simulink model "topology"  (R2024b)
settings: Solver=FixedStepDiscrete  StartTime=0.0  StopTime=0.2  FixedStep=1e-6  MaxStep=1e-6  RelTol=1e-6
libraries: spsMosfetLib x16, spsSeriesRLCBranchLib x16, spsIdealSwitchLib x10, simulink x7, spsVoltageMeasurementLib x6, spsCurrentMeasurementLib x5, spsDCVoltageSourceLib x4, spsACVoltageSourceLib x1, sps_lib x1
settings Model: DataDictionary=CHB_Data.sldd  Creator=licuiting  LastModifiedBy=licuiting
settings SolverCC: InitialStep=1e-6
settings ModelReferenceCC: ModelReferenceNumInstancesAllowed=Single

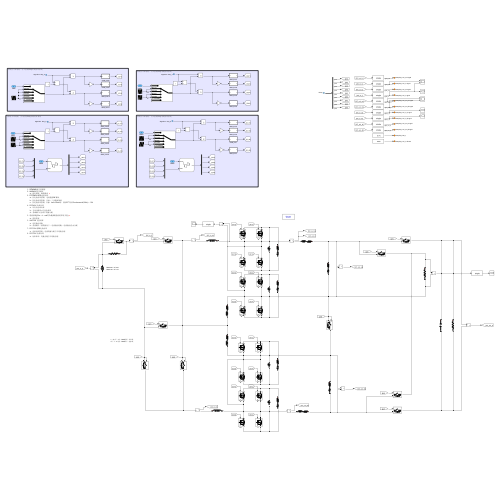
[thumbnail: Simulink's stored preview of the top-level diagram]
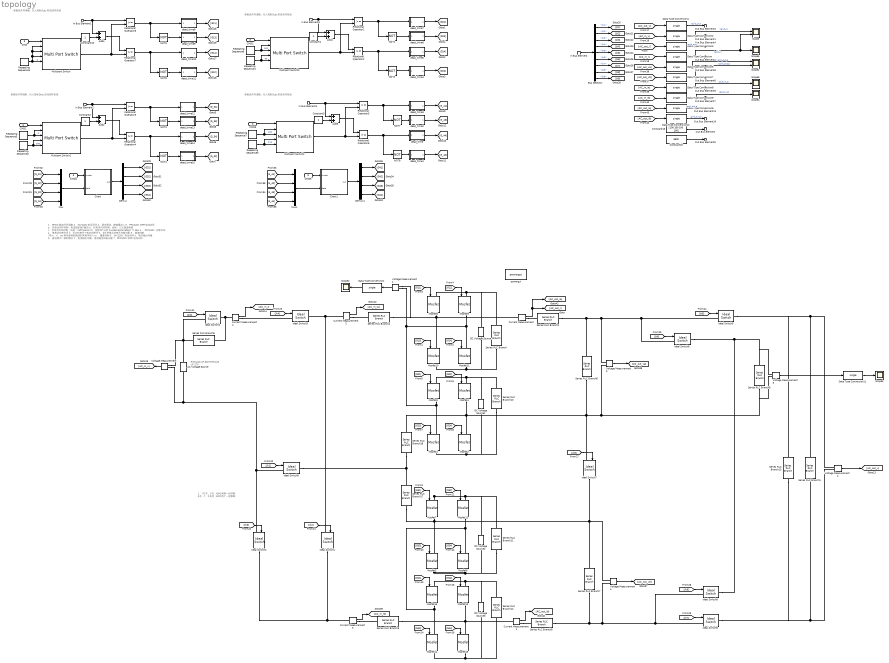
== system topology ==
  note: RMS:240   UF:340
      | RMS:120   UF:170
  note: 1、SPWM载波开环调制
      | 2、INV240V电压闭环
      | a、逐步限流、峰值限流 x
      | 3、PFC240V QPR电流内环
      | a、仅电流内环控制：电流超前90°解决
      | b、仅电流内环控制：目标：三次谐波削弱
      | c、仅电流内环控制：目标：Iref=15cos时，实际FFT分析 Fundamental(50Hz) = 15A
      | 4、PFC240V 功率外环
      | a、单有功功率外环
      | b、无功功率环+有功功率环
      | d、各H桥单元功率不均衡分配
      | 5、谐波抑制 (带rc、rl、rcd等负载抑制谐波的常用手段) x
      | a、 重复控制
      | 6、INV120V 电压闭环
      | a、电压输出均衡
      | b、直流源不一致的情况下，电流输出均衡，电流输出自由分配
      | 7、PFC120V QPR电流内环
      | a、电流内环控制，电流均衡分配与不均衡分配
      | 8、PFC120V 功率外环
      | a、功率外环，均衡分配与不均衡分配
  note: 1、2打开，3关，BMS两两一组并联
      | 3开，1、2关闭，BMS四个一起串联
  note: 单极性开环调制，引入控制Duty形成闭环系统
  note: 单极性开环调制，引入控制Duty形成闭环系统
  note: 单极性开环调制，引入控制Duty形成闭环系统
  note: 单极性开环调制，引入控制Duty形成闭环系统
  In Bus Element : Inport  PortName=Relay
  In Bus Element1 : Inport  Port=2  PortName=Algorithm  Element=duty_a
  In Bus Element3 : Inport  Port=2  PortName=Algorithm  Element=duty_a
  In Bus Element2 : Inport  Port=2  PortName=Algorithm  Element=duty_b
  In Bus Element4 : Inport  Port=2  PortName=Algorithm  Element=duty_b
  CMD : Inport  Port=3  OutDataTypeStr=Enum: CHB_MODE
  AC Voltage Source : spsACVoltageSourceLib/AC Voltage Source  Amplitude=170  Phase=0  Frequency=50  SampleTime=0  Measurements=None  BusType=swing  Pref=10e3  Qref=0  Qmin=-inf  Qmax=+inf
  Add{1..4} (4 alike) : Sum
  Bus Selector : BusSelector  OutputSignals=jk1,jk2,jk3,jk4,jk5,jk6,jk7,jk8,jk9
  CMD{1..5} (5 alike) : InportShadow  Port=3  OutDataTypeStr=Enum: CHB_MODE
  Chart : Stateflow chart  TreatAsAtomicUnit=on
  Chart1 : Stateflow chart  TreatAsAtomicUnit=on
  Constant{1..3,10} (4 alike) : Constant
  Constant16 : Constant  Value=[100 100 100 100]  OutDataTypeStr=single
  Constant20 : Constant  Value=3600  OutDataTypeStr=single
  Current Measurement{,1..4} (5 alike) : spsCurrentMeasurementLib/Current Measurement  PhasorSimulation=off  OutputType=Complex  PSBequivalent=0
  DC Voltage Source{,1..3} (4 alike) : spsDCVoltageSourceLib/DC Voltage Source  Amplitude=100  Measurements=None
  Data Type Conversion{,1..11} (12 alike) : DataTypeConversion  OutDataTypeStr=single  SaturateOnIntegerOverflow=off  RndMeth=Floor
  Demux : Demux
  Demux1 : Demux
  Ideal Switch{0..9} (10 alike) : spsIdealSwitchLib/Ideal Switch  Ron=0.001  Lon=0  IC=0  Rs=1e5  Cs=inf  Measurements=off
  Mosfet{1..16} (16 alike) : spsMosfetLib/Mosfet  Ron=0.01  Lon=0  Rd=0.01  Vfd=0  IC=0  Rs=1e5  Cs=inf  Measurements=on
  Multiport Switch{,1..3} (4 alike) : MultiPortSwitch  DataPortOrder=Specify indices  Inputs=4  DataPortIndices={CHB_MODE.INV120,CHB_MODE.PFC120,CHB_MODE.INV240,CHB_MODE.PFC240,CHB_MODE.STANDBY}  OutDataTypeStr=single  SaturateOnIntegerOverflow=off  InputSameDT=off
  Mux : Mux
  Mux1 : Mux
  NOT{1..8} (8 alike) : Logic  Operator=NOT  IconShape=distinctive  AllPortsSameDT=off  OutDataTypeStr=boolean
  Relational Operator{1..8} (8 alike) : RelationalOperator  OutDataTypeStr=boolean  RndMeth=Simplest  InputSameDT=off
  Repeating Sequence1 : simulink/Sources/Repeating Sequence  rep_seq_t=[0 2.5e-5 7.5e-5 1e-4]  rep_seq_y=[0.5 1 0 0.5]
  Repeating Sequence2 : simulink/Sources/Repeating Sequence  rep_seq_t=[0 5e-5 1e-4]  rep_seq_y=[0 1 0]
  Repeating Sequence3 : simulink/Sources/Repeating Sequence  rep_seq_t=[0 2.5e-5 7.5e-5 1e-4]  rep_seq_y=[0.5 0 1 0.5]
  Repeating Sequence4 : simulink/Sources/Repeating Sequence  rep_seq_t=[0 5e-5 1e-4]  rep_seq_y=[1 0 1]
  Repeating Sequence5 : simulink/Sources/Repeating Sequence  rep_seq_t=[0 5e-5 1e-4]  rep_seq_y=[1 0 1]
  Repeating Sequence6 : simulink/Sources/Repeating Sequence  rep_seq_t=[0 5e-5 1e-4]  rep_seq_y=[0 1 0]
  Repeating Sequence7 : simulink/Sources/Repeating Sequence  rep_seq_t=[0 5e-5 1e-4]  rep_seq_y=[0 1 0]
  Scope : Scope  NumInputPorts=2
  Scope1 : Scope  NumInputPorts=2
  Scope{2..6} (5 alike) : Scope
  Series RLC Branch{,10..12} (4 alike) : spsSeriesRLCBranchLib/Series RLC Branch  LConnTagsString=__new0  RConnTagsString=__new0  BranchType=RC  Resistance=0.5  Inductance=1e-3  SetiL0=off  InitialCurrent=0  Capacitance=4.7e-6  Setx0=off  InitialVoltage=0  Measurements=None
  Series RLC Branch1 : spsSeriesRLCBranchLib/Series RLC Branch  LConnTagsString=__new0  RConnTagsString=__new0  BranchType=R  Resistance=100  Inductance=1e-3  SetiL0=off  InitialCurrent=0  Capacitance=1e-6  Setx0=off  InitialVoltage=0  Measurements=None
  Series RLC Branch13 : spsSeriesRLCBranchLib/Series RLC Branch  LConnTagsString=__new0  RConnTagsString=__new0  BranchType=C  Resistance=100  Inductance=1e-3  SetiL0=off  InitialCurrent=0  Capacitance=4.2e-6  Setx0=off  InitialVoltage=0  Measurements=None
  Series RLC Branch{2,9,17..18} (4 alike) : spsSeriesRLCBranchLib/Series RLC Branch  LConnTagsString=__new0  RConnTagsString=__new0  BranchType=RL  Resistance=0.2  Inductance=1e-3  SetiL0=off  InitialCurrent=0  Capacitance=1e-6  Setx0=off  InitialVoltage=0  Measurements=None
  Series RLC Branch3 : spsSeriesRLCBranchLib/Series RLC Branch  LConnTagsString=__new0  RConnTagsString=__new0  BranchType=L  Resistance=0.2  Inductance=1e-3  SetiL0=off  InitialCurrent=0  Capacitance=1e-6  Setx0=off  InitialVoltage=0  Measurements=None
  Series RLC Branch4 : spsSeriesRLCBranchLib/Series RLC Branch  LConnTagsString=__new0  RConnTagsString=__new0  BranchType=L  Resistance=0.2  Inductance=1e-3  SetiL0=off  InitialCurrent=0  Capacitance=1e-6  Setx0=off  InitialVoltage=0  Measurements=None
  Series RLC Branch5 : spsSeriesRLCBranchLib/Series RLC Branch  LConnTagsString=__new0  RConnTagsString=__new0  BranchType=R  Resistance=0.2  Inductance=2e-3  SetiL0=off  InitialCurrent=0  Capacitance=1e-6  Setx0=off  InitialVoltage=0  Measurements=None
  Series RLC Branch6 : spsSeriesRLCBranchLib/Series RLC Branch  LConnTagsString=__new0  RConnTagsString=__new0  BranchType=RC  Resistance=0.2  Inductance=1e-3  SetiL0=off  InitialCurrent=0  Capacitance=4.2e-6  Setx0=off  InitialVoltage=0  Measurements=None
  Series RLC Branch7 : spsSeriesRLCBranchLib/Series RLC Branch  LConnTagsString=__new0  RConnTagsString=__new0  BranchType=RC  Resistance=0.2  Inductance=1e-3  SetiL0=off  InitialCurrent=0  Capacitance=4.2e-6  Setx0=off  InitialVoltage=0  Measurements=None
  Series RLC Branch8 : spsSeriesRLCBranchLib/Series RLC Branch  LConnTagsString=__new0  RConnTagsString=__new0  BranchType=R  Resistance=5  Inductance=1e-3  SetiL0=off  InitialCurrent=0  Capacitance=1e-6  Setx0=off  InitialVoltage=0  Measurements=None
  Voltage Measurement{,1..5} (6 alike) : spsVoltageMeasurementLib/Voltage Measurement  PhasorSimulation=off  OutputType=Complex  PSBequivalent=0
  dead_time : Subsystem  TreatAsAtomicUnit=on
  dead_time1 : Subsystem  TreatAsAtomicUnit=on
  dead_time10 : Subsystem  TreatAsAtomicUnit=on
  dead_time11 : Subsystem  TreatAsAtomicUnit=on
  dead_time12 : Subsystem  TreatAsAtomicUnit=on
  dead_time13 : Subsystem  TreatAsAtomicUnit=on
  dead_time14 : Subsystem  TreatAsAtomicUnit=on
  dead_time15 : Subsystem  TreatAsAtomicUnit=on
  dead_time2 : Subsystem  TreatAsAtomicUnit=on
  dead_time3 : Subsystem  TreatAsAtomicUnit=on
  dead_time4 : Subsystem  TreatAsAtomicUnit=on
  dead_time5 : Subsystem  TreatAsAtomicUnit=on
  dead_time6 : Subsystem  TreatAsAtomicUnit=on
  dead_time7 : Subsystem  TreatAsAtomicUnit=on
  dead_time8 : Subsystem  TreatAsAtomicUnit=on
  dead_time9 : Subsystem  TreatAsAtomicUnit=on
  powergui : sps_lib/powergui  Priority=1  SimulationMode=Discrete  SampleTime=1e-6  frequency=60  Iterations=50  frequencyindice=0  Pbase=100e6  ErrMax=1e-4  UnitsV=kV  UnitsW=MW  buscounter=0  FunctionMessages=off  echomessages=off  EnableUseOfTLC=off  CurrentSourceSwitches=off  DisableSnubberDevices=off  DisableRonSwitches=off  DisableVfSwitches=off  DisplayEquations=off  AutomaticDiscreteSolvers=off  SolverType=Tustin/Backward Euler (TBE)  Interpol=off  ExternalGateDelay=off  methode=off  Ts=100  x0status=blocks  SPID=on  SwTol=0  HookPort=off  NonlinearTolerance=1e-4  nMaxIteration=100  ContinueOnMaxIteration=off  RestoreLinks=warning  ResistiveCurrentMeasurement=off  Frange=[0:2:500]  Ylog=off  Xlog=on  ShowGrid=off  save=off  variable=ZData  structure=0  ZoomFFT=off  StartTime=0.0  cycles=1  DisplayStyle=1  fundamental=60  FreqAxis=off  MaxFrequency=1000  frequencyindicesteady=1  RmsSteady=1  display=off
  Out Bus Element1 : Outport  PortName=Sampling  Element=AC_in.Vgrid
  Out Bus Element2 : Outport  PortName=Sampling  Element=AC_in.Igrid
  Out Bus Element5 : Outport  PortName=Sampling  Element=AC_in.Power
  Out Bus Element3 : Outport  PortName=Sampling  Element=AC_out.Vgrid
  Out Bus Element4 : Outport  PortName=Sampling  Element=AC_out.Igrid
  Out Bus Element8 : Outport  PortName=Sampling  Element=AC_out_A.Vgrid
  Out Bus Element11 : Outport  PortName=Sampling  Element=AC_out_A.Igrid
  Out Bus Element6 : Outport  PortName=Sampling  Element=AC_out_B.Vgrid
  Out Bus Element10 : Outport  PortName=Sampling  Element=AC_out_B.Igrid
  Out Bus Element9 : Outport  PortName=Sampling  Element=AC_in_A.Igrid
  Out Bus Element7 : Outport  PortName=Sampling  Element=AC_in_B.Igrid
  Out Bus Element : Outport  PortName=Sampling  Element=bat_v
  wires:
  Relational Operator6/1 -> dead_time8/1(Input), NOT5/1
  Add4/1 -> Relational Operator7/1
  Constant10/1 -> Add4/2
  Relational Operator2/1 -> dead_time5/1(Input), NOT2/1
  Constant1/1 -> Add1/2
  Add1/1 -> Relational Operator2/1
  Relational Operator1/1 -> dead_time7/1(Input), NOT1/1
  Relational Operator3/1 -> dead_time12/1(Input), NOT3/1
  Add2/1 -> Relational Operator4/1
  Constant2/1 -> Add2/2
  Relational Operator4/1 -> dead_time14/1(Input), NOT4/1
  Relational Operator8/1 -> dead_time/1(Input), NOT8/1
  Constant3/1 -> Add3/2
  Add3/1 -> Relational Operator8/1
  Relational Operator5/1 -> dead_time3/1(Input), NOT7/1
  [G14] -> Mosfet11/1
  [G13] -> Mosfet10/1
  [G11] -> Mosfet8/1
  [G12] -> Mosfet9/1
  [G21] -> Mosfet3/1
  [G22] -> Mosfet4/1
  [G23] -> Mosfet1/1
  [G24] -> Mosfet2/1
  [G31] -> Mosfet7/1
  [G34] -> Mosfet6/1
  [G41] -> Mosfet16/1
  [G44] -> Mosfet15/1
  Relational Operator7/1 -> dead_time10/1(Input), NOT6/1
  [G33] -> Mosfet5/1
  [G32] -> Mosfet12/1
  [G43] -> Mosfet14/1
  [G42] -> Mosfet13/1
  Data Type Conversion1/1 -> Scope2/1
  Voltage Measurement1/1 -> Data Type Conversion1/1
  Voltage Measurement/1 -> [AC_in_v]
  Current Measurement/1 -> [AC_out_i], [AC_out_ia]
  [AC_out_v] -> Data Type Conversion4/1
  [AC_in_i] -> Data Type Conversion/1
  [AC_in_v] -> Data Type Conversion2/1
  [AC_out_i] -> Data Type Conversion3/1
  In Bus Element/1 -> Bus Selector/1
  Bus Selector/1 -> [jk1]  "<jk1>"
  Bus Selector/2 -> [jk2]  "<jk2>"
  Bus Selector/3 -> [jk3]  "<jk3>"
  Bus Selector/4 -> [jk4]  "<jk4>"
  Bus Selector/5 -> [jk5]  "<jk5>"
  Bus Selector/6 -> [jk6]  "<jk6>"
  Bus Selector/7 -> [jk7]  "<jk7>"
  Bus Selector/8 -> [jk8]  "<jk8>"
  Constant16/1 -> Out Bus Element/1
  Data Type Conversion2/1 -> Scope/1, Out Bus Element1/1  "Vgrid_in"
  Data Type Conversion/1 -> Scope/2, Scope5/1, Out Bus Element2/1  "Igrid_in"
  Data Type Conversion4/1 -> Out Bus Element3/1  "Vgrid_out"
  Data Type Conversion3/1 -> Out Bus Element4/1  "Igrid_out"
  Voltage Measurement2/1 -> [AC_out_v]
  [jk4] -> Ideal Switch3/1
  [jk1] -> Ideal Switch0/1
  [jk3] -> Ideal Switch2/1
  [jk2] -> Ideal Switch1/1
  [jk6] -> Ideal Switch6/1
  [jk8] -> Ideal Switch7/1
  [jk5] -> Ideal Switch5/1
  Constant20/1 -> Out Bus Element5/1
  CMD/1 -> Multiport Switch/1
  Multiport Switch3/1 -> Relational Operator1/2, Relational Operator2/2
  Multiport Switch2/1 -> Relational Operator5/2, Relational Operator8/2
  Multiport Switch/1 -> Relational Operator6/2, Relational Operator7/2
  Repeating Sequence2/1 -> Multiport Switch1/4, Multiport Switch1/5  "180"
  Repeating Sequence4/1 -> Multiport Switch/3, Multiport Switch/2, Multiport Switch/4, Multiport Switch/5  "0"
  Repeating Sequence1/1 -> Multiport Switch3/4, Multiport Switch3/5  "90"
  Repeating Sequence3/1 -> Multiport Switch2/4, Multiport Switch2/5  "270"
  CMD1/1 -> Multiport Switch1/1
  CMD3/1 -> Multiport Switch2/1
  CMD2/1 -> Multiport Switch3/1
  Repeating Sequence5/1 -> Multiport Switch1/2, Multiport Switch1/3  "0"
  Repeating Sequence6/1 -> Multiport Switch3/2, Multiport Switch3/3  "180"
  Repeating Sequence7/1 -> Multiport Switch2/3, Multiport Switch2/2  "180"
  [jk7] -> Ideal Switch9/1
  Bus Selector/9 -> [jk9]  "<jk9>"
  [jk9] -> Ideal Switch8/1
  Multiport Switch1/1 -> Relational Operator3/2, Relational Operator4/2
  [G_34] -> Mux/4
  [G_33] -> Mux/3
  [G_32] -> Mux/2
  [G_31] -> Mux/1
  Mux/1 -> Chart/2(data)
  CMD4/1 -> Chart/1(mode)
  Chart/1(out) -> Demux/1
  Demux/1 -> [G31]
  Demux/2 -> [G32]
  Demux/3 -> [G33]
  Demux/4 -> [G34]
  Mux1/1 -> Chart1/2(data)
  [G_41] -> Mux1/1
  [G_42] -> Mux1/2
  [G_43] -> Mux1/3
  [G_44] -> Mux1/4
  CMD5/1 -> Chart1/1(mode)
  Chart1/1(out) -> Demux1/1
  Demux1/1 -> [G41]
  Demux1/2 -> [G42]
  Demux1/3 -> [G43]
  Demux1/4 -> [G44]
  [AC_out_vb] -> Data Type Conversion7/1
  [AC_out_va] -> Data Type Conversion5/1
  Data Type Conversion7/1 -> Scope1/2, Out Bus Element6/1  "vgrid_out_b"
  Data Type Conversion5/1 -> Scope1/1, Out Bus Element8/1  "vgrid_out_a"
  Data Type Conversion9/1 -> Out Bus Element7/1, Scope4/1  "igrid_in_b"
  Data Type Conversion8/1 -> Out Bus Element9/1, Scope6/1  "igrid_in_a"
  In Bus Element1/1 -> Relational Operator6/1, Add4/1
  In Bus Element3/1 -> Add1/1, Relational Operator1/1
  In Bus Element4/1 -> Add3/1, Relational Operator5/1
  In Bus Element2/1 -> Add2/1, Relational Operator3/1
  [AC_in_ia] -> Data Type Conversion8/1
  [AC_in_ib] -> Data Type Conversion9/1
  Current Measurement2/1 -> [AC_in_ia]
  Current Measurement3/1 -> [AC_in_ib]
  Current Measurement4/1 -> [AC_in_i]
  [jk2] -> Ideal Switch4/1
  Data Type Conversion6/1 -> Out Bus Element11/1  "igrid_out_a"
  Data Type Conversion10/1 -> Out Bus Element10/1  "igrid_out_b"
  [AC_out_ia] -> Data Type Conversion6/1
  [AC_out_ib] -> Data Type Conversion10/1
  Current Measurement1/1 -> [AC_out_ib]
  Voltage Measurement3/1 -> [AC_out_va]
  Voltage Measurement4/1 -> [AC_out_vb]
  Voltage Measurement5/1 -> Data Type Conversion11/1
  Data Type Conversion11/1 -> Scope3/1
  NOT5/1 -> dead_time9/1(Input)
  NOT6/1 -> dead_time11/1(Input)
  dead_time8/1(Out1) -> [G11]
  dead_time9/1(Out1) -> [G13]
  dead_time10/1(Out1) -> [G14]
  dead_time11/1(Out1) -> [G12]
  NOT1/1 -> dead_time6/1(Input)
  NOT2/1 -> dead_time4/1(Input)
  dead_time7/1(Out1) -> [G21]
  dead_time6/1(Out1) -> [G23]
  dead_time5/1(Out1) -> [G24]
  dead_time4/1(Out1) -> [G22]
  dead_time3/1(Out1) -> [G_41]
  dead_time2/1(Out1) -> [G_43]
  dead_time/1(Out1) -> [G_44]
  dead_time1/1(Out1) -> [G_42]
  NOT8/1 -> dead_time1/1(Input)
  NOT7/1 -> dead_time2/1(Input)
  dead_time14/1(Out1) -> [G_34]
  dead_time13/1(Out1) -> [G_33]
  dead_time12/1(Out1) -> [G_31]
  dead_time15/1(Out1) -> [G_32]
  NOT4/1 -> dead_time15/1(Input)
  NOT3/1 -> dead_time13/1(Input)
  connections:
  Mosfet9/LConn1 -- DC Voltage Source/RConn1 -- Series RLC Branch/LConn1 -- Mosfet8/LConn1
  Mosfet11/RConn1 -- Series RLC Branch/RConn1 -- DC Voltage Source/LConn1 -- Mosfet10/RConn1
  Mosfet4/LConn1 -- Series RLC Branch10/LConn1 -- DC Voltage Source1/RConn1 -- Mosfet3/LConn1
  Mosfet2/RConn1 -- Series RLC Branch10/RConn1 -- DC Voltage Source1/LConn1 -- Mosfet1/RConn1
  Mosfet9/RConn1 -- Mosfet11/LConn1 -- Voltage Measurement1/LConn1 -- Mosfet3/RConn1 -- Mosfet1/LConn1
  Mosfet7/LConn1 -- Series RLC Branch11/LConn1 -- DC Voltage Source2/RConn1 -- Mosfet12/LConn1
  Mosfet5/RConn1 -- Series RLC Branch11/RConn1 -- DC Voltage Source2/LConn1 -- Mosfet6/RConn1
  Mosfet13/LConn1 -- Series RLC Branch12/LConn1 -- DC Voltage Source3/RConn1 -- Mosfet16/LConn1
  Mosfet15/RConn1 -- Series RLC Branch12/RConn1 -- DC Voltage Source3/LConn1 -- Mosfet14/RConn1
  Ideal Switch2/RConn1 -- Current Measurement3/LConn1 -- Ideal Switch1/RConn1
  Ideal Switch2/LConn1 -- Voltage Measurement/LConn2 -- AC Voltage Source/LConn1 -- Ideal Switch0/LConn1
  Voltage Measurement/LConn1 -- Ideal Switch4/LConn1 -- AC Voltage Source/RConn1 -- Series RLC Branch5/RConn1
  Voltage Measurement2/LConn1 -- Series RLC Branch13/LConn1 -- Ideal Switch5/RConn1 -- Series RLC Branch1/LConn1
  Series RLC Branch2/LConn1 -- Voltage Measurement3/LConn1 -- Ideal Switch6/LConn1 -- Ideal Switch5/LConn1 -- Series RLC Branch6/LConn1
  Mosfet12/RConn1 -- Mosfet6/LConn1 -- Mosfet16/RConn1 -- Mosfet14/LConn1
  Ideal Switch6/RConn1 -- Series RLC Branch8/LConn1 -- Voltage Measurement5/LConn1 -- Ideal Switch8/RConn1
  Voltage Measurement2/LConn2 -- Ideal Switch9/RConn1 -- Series RLC Branch13/RConn1 -- Series RLC Branch1/RConn1
  Current Measurement/RConn1 -- Series RLC Branch2/RConn1
  Ideal Switch4/RConn1 -- Current Measurement4/LConn1 -- Series RLC Branch5/LConn1
  Series RLC Branch17/RConn1 -- Mosfet5/LConn1 -- Series RLC Branch7/LConn1 -- Voltage Measurement4/LConn2 -- Ideal Switch7/RConn1 -- Mosfet7/RConn1
  Series RLC Branch6/RConn1 -- Series RLC Branch8/RConn1 -- Voltage Measurement5/LConn2 -- Voltage Measurement3/LConn2 -- Ideal Switch7/LConn1 -- Mosfet4/RConn1 -- Series RLC Branch18/LConn1 -- Mosfet2/LConn1
  Series RLC Branch18/RConn1 -- Ideal Switch0/RConn1 -- Series RLC Branch17/LConn1
  Series RLC Branch7/RConn1 -- Series RLC Branch9/LConn1 -- Voltage Measurement4/LConn1 -- Ideal Switch9/LConn1 -- Ideal Switch8/LConn1
  Mosfet8/RConn1 -- Series RLC Branch4/LConn1 -- Voltage Measurement1/LConn2 -- Current Measurement/LConn1 -- Mosfet10/LConn1
  Current Measurement2/LConn1 -- Ideal Switch3/RConn1 -- Ideal Switch1/LConn1
  Mosfet13/RConn1 -- Mosfet15/LConn1 -- Series RLC Branch3/RConn1 -- Current Measurement1/LConn1
  Current Measurement3/RConn1 -- Series RLC Branch3/LConn1
  Current Measurement2/RConn1 -- Series RLC Branch4/RConn1
  Current Measurement4/RConn1 -- Ideal Switch3/LConn1
  Current Measurement1/RConn1 -- Series RLC Branch9/RConn1

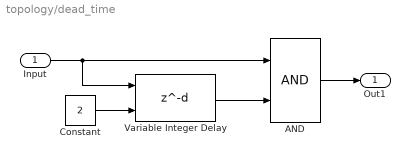
== system topology/dead_time ==
  Input : Inport  OutDataTypeStr=boolean
  AND : Logic  IconShape=distinctive  AllPortsSameDT=off  OutDataTypeStr=boolean
  Constant : Constant  Value=2  OutDataTypeStr=uint32
  Variable Integer Delay : Delay  DelayLengthSource=Input port  DelayLengthUpperLimit=10
      settings: InputPortMap=u0,p1
  Out1 : Outport  OutDataTypeStr=boolean
  wires:
  Constant/1 -> Variable Integer Delay/2
  AND/1 -> Out1/1
  Variable Integer Delay/1 -> AND/2
  Input/1 -> Variable Integer Delay/1, AND/1

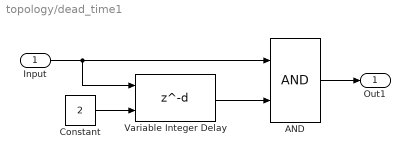
== system topology/dead_time1 ==
  Input : Inport  OutDataTypeStr=boolean
  AND : Logic  IconShape=distinctive  AllPortsSameDT=off  OutDataTypeStr=boolean
  Constant : Constant  Value=2  OutDataTypeStr=uint32
  Variable Integer Delay : Delay  DelayLengthSource=Input port  DelayLengthUpperLimit=10
      settings: InputPortMap=u0,p1
  Out1 : Outport  OutDataTypeStr=boolean
  wires:
  Input/1 -> AND/1, Variable Integer Delay/1
  Variable Integer Delay/1 -> AND/2
  AND/1 -> Out1/1
  Constant/1 -> Variable Integer Delay/2

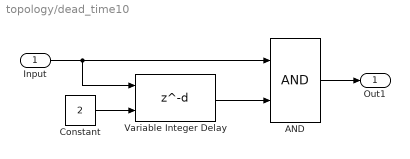
== system topology/dead_time10 ==
  Input : Inport  OutDataTypeStr=boolean
  AND : Logic  IconShape=distinctive  AllPortsSameDT=off  OutDataTypeStr=boolean
  Constant : Constant  Value=2  OutDataTypeStr=uint32
  Variable Integer Delay : Delay  DelayLengthSource=Input port  DelayLengthUpperLimit=10
      settings: InputPortMap=u0,p1
  Out1 : Outport  OutDataTypeStr=boolean
  wires:
  Input/1 -> AND/1, Variable Integer Delay/1
  Variable Integer Delay/1 -> AND/2
  AND/1 -> Out1/1
  Constant/1 -> Variable Integer Delay/2

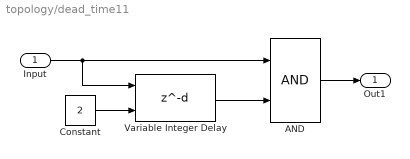
== system topology/dead_time11 ==
  Input : Inport  OutDataTypeStr=boolean
  AND : Logic  IconShape=distinctive  AllPortsSameDT=off  OutDataTypeStr=boolean
  Constant : Constant  Value=2  OutDataTypeStr=uint32
  Variable Integer Delay : Delay  DelayLengthSource=Input port  DelayLengthUpperLimit=10
      settings: InputPortMap=u0,p1
  Out1 : Outport  OutDataTypeStr=boolean
  wires:
  Constant/1 -> Variable Integer Delay/2
  AND/1 -> Out1/1
  Variable Integer Delay/1 -> AND/2
  Input/1 -> Variable Integer Delay/1, AND/1

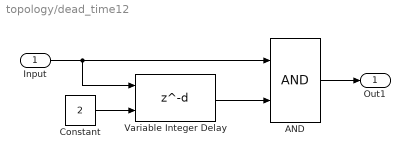
== system topology/dead_time12 ==
  Input : Inport  OutDataTypeStr=boolean
  AND : Logic  IconShape=distinctive  AllPortsSameDT=off  OutDataTypeStr=boolean
  Constant : Constant  Value=2  OutDataTypeStr=uint32
  Variable Integer Delay : Delay  DelayLengthSource=Input port  DelayLengthUpperLimit=10
      settings: InputPortMap=u0,p1
  Out1 : Outport  OutDataTypeStr=boolean
  wires:
  Input/1 -> AND/1, Variable Integer Delay/1
  Variable Integer Delay/1 -> AND/2
  AND/1 -> Out1/1
  Constant/1 -> Variable Integer Delay/2

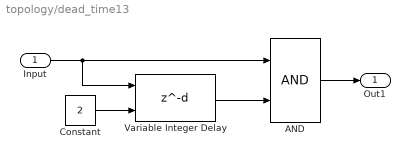
== system topology/dead_time13 ==
  Input : Inport  OutDataTypeStr=boolean
  AND : Logic  IconShape=distinctive  AllPortsSameDT=off  OutDataTypeStr=boolean
  Constant : Constant  Value=2  OutDataTypeStr=uint32
  Variable Integer Delay : Delay  DelayLengthSource=Input port  DelayLengthUpperLimit=10
      settings: InputPortMap=u0,p1
  Out1 : Outport  OutDataTypeStr=boolean
  wires:
  Constant/1 -> Variable Integer Delay/2
  AND/1 -> Out1/1
  Variable Integer Delay/1 -> AND/2
  Input/1 -> Variable Integer Delay/1, AND/1

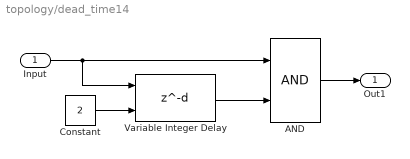
== system topology/dead_time14 ==
  Input : Inport  OutDataTypeStr=boolean
  AND : Logic  IconShape=distinctive  AllPortsSameDT=off  OutDataTypeStr=boolean
  Constant : Constant  Value=2  OutDataTypeStr=uint32
  Variable Integer Delay : Delay  DelayLengthSource=Input port  DelayLengthUpperLimit=10
      settings: InputPortMap=u0,p1
  Out1 : Outport  OutDataTypeStr=boolean
  wires:
  Input/1 -> AND/1, Variable Integer Delay/1
  Variable Integer Delay/1 -> AND/2
  AND/1 -> Out1/1
  Constant/1 -> Variable Integer Delay/2

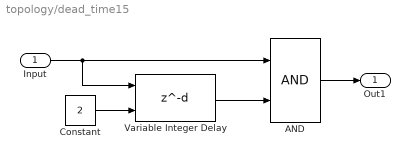
== system topology/dead_time15 ==
  Input : Inport  OutDataTypeStr=boolean
  AND : Logic  IconShape=distinctive  AllPortsSameDT=off  OutDataTypeStr=boolean
  Constant : Constant  Value=2  OutDataTypeStr=uint32
  Variable Integer Delay : Delay  DelayLengthSource=Input port  DelayLengthUpperLimit=10
      settings: InputPortMap=u0,p1
  Out1 : Outport  OutDataTypeStr=boolean
  wires:
  Constant/1 -> Variable Integer Delay/2
  AND/1 -> Out1/1
  Variable Integer Delay/1 -> AND/2
  Input/1 -> Variable Integer Delay/1, AND/1

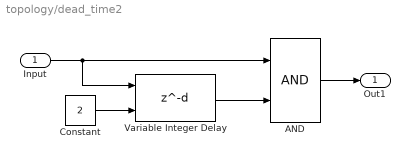
== system topology/dead_time2 ==
  Input : Inport  OutDataTypeStr=boolean
  AND : Logic  IconShape=distinctive  AllPortsSameDT=off  OutDataTypeStr=boolean
  Constant : Constant  Value=2  OutDataTypeStr=uint32
  Variable Integer Delay : Delay  DelayLengthSource=Input port  DelayLengthUpperLimit=10
      settings: InputPortMap=u0,p1
  Out1 : Outport  OutDataTypeStr=boolean
  wires:
  Input/1 -> AND/1, Variable Integer Delay/1
  Variable Integer Delay/1 -> AND/2
  AND/1 -> Out1/1
  Constant/1 -> Variable Integer Delay/2

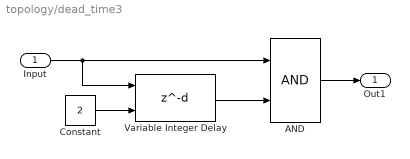
== system topology/dead_time3 ==
  Input : Inport  OutDataTypeStr=boolean
  AND : Logic  IconShape=distinctive  AllPortsSameDT=off  OutDataTypeStr=boolean
  Constant : Constant  Value=2  OutDataTypeStr=uint32
  Variable Integer Delay : Delay  DelayLengthSource=Input port  DelayLengthUpperLimit=10
      settings: InputPortMap=u0,p1
  Out1 : Outport  OutDataTypeStr=boolean
  wires:
  Constant/1 -> Variable Integer Delay/2
  AND/1 -> Out1/1
  Variable Integer Delay/1 -> AND/2
  Input/1 -> Variable Integer Delay/1, AND/1

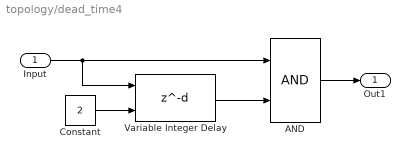
== system topology/dead_time4 ==
  Input : Inport  OutDataTypeStr=boolean
  AND : Logic  IconShape=distinctive  AllPortsSameDT=off  OutDataTypeStr=boolean
  Constant : Constant  Value=2  OutDataTypeStr=uint32
  Variable Integer Delay : Delay  DelayLengthSource=Input port  DelayLengthUpperLimit=10
      settings: InputPortMap=u0,p1
  Out1 : Outport  OutDataTypeStr=boolean
  wires:
  Input/1 -> AND/1, Variable Integer Delay/1
  Variable Integer Delay/1 -> AND/2
  AND/1 -> Out1/1
  Constant/1 -> Variable Integer Delay/2

== system topology/dead_time5 ==
  Input : Inport  OutDataTypeStr=boolean
  AND : Logic  IconShape=distinctive  AllPortsSameDT=off  OutDataTypeStr=boolean
  Constant : Constant  Value=2  OutDataTypeStr=uint32
  Variable Integer Delay : Delay  DelayLengthSource=Input port  DelayLengthUpperLimit=10
      settings: InputPortMap=u0,p1
  Out1 : Outport  OutDataTypeStr=boolean
  wires:
  Constant/1 -> Variable Integer Delay/2
  AND/1 -> Out1/1
  Variable Integer Delay/1 -> AND/2
  Input/1 -> Variable Integer Delay/1, AND/1

== system topology/dead_time6 ==
  Input : Inport  OutDataTypeStr=boolean
  AND : Logic  IconShape=distinctive  AllPortsSameDT=off  OutDataTypeStr=boolean
  Constant : Constant  Value=2  OutDataTypeStr=uint32
  Variable Integer Delay : Delay  DelayLengthSource=Input port  DelayLengthUpperLimit=10
      settings: InputPortMap=u0,p1
  Out1 : Outport  OutDataTypeStr=boolean
  wires:
  Input/1 -> AND/1, Variable Integer Delay/1
  Variable Integer Delay/1 -> AND/2
  AND/1 -> Out1/1
  Constant/1 -> Variable Integer Delay/2

== system topology/dead_time7 ==
  Input : Inport  OutDataTypeStr=boolean
  AND : Logic  IconShape=distinctive  AllPortsSameDT=off  OutDataTypeStr=boolean
  Constant : Constant  Value=2  OutDataTypeStr=uint32
  Variable Integer Delay : Delay  DelayLengthSource=Input port  DelayLengthUpperLimit=10
      settings: InputPortMap=u0,p1
  Out1 : Outport  OutDataTypeStr=boolean
  wires:
  Constant/1 -> Variable Integer Delay/2
  AND/1 -> Out1/1
  Variable Integer Delay/1 -> AND/2
  Input/1 -> Variable Integer Delay/1, AND/1

== system topology/dead_time8 ==
  Input : Inport  OutDataTypeStr=boolean
  AND : Logic  IconShape=distinctive  AllPortsSameDT=off  OutDataTypeStr=boolean
  Constant : Constant  Value=2  OutDataTypeStr=uint32
  Variable Integer Delay : Delay  DelayLengthSource=Input port  DelayLengthUpperLimit=10
      settings: InputPortMap=u0,p1
  Out1 : Outport  OutDataTypeStr=boolean
  wires:
  Input/1 -> AND/1, Variable Integer Delay/1
  Variable Integer Delay/1 -> AND/2
  AND/1 -> Out1/1
  Constant/1 -> Variable Integer Delay/2

== system topology/dead_time9 ==
  Input : Inport  OutDataTypeStr=boolean
  AND : Logic  IconShape=distinctive  AllPortsSameDT=off  OutDataTypeStr=boolean
  Constant : Constant  Value=2  OutDataTypeStr=uint32
  Variable Integer Delay : Delay  DelayLengthSource=Input port  DelayLengthUpperLimit=10
      settings: InputPortMap=u0,p1
  Out1 : Outport  OutDataTypeStr=boolean
  wires:
  Constant/1 -> Variable Integer Delay/2
  AND/1 -> Out1/1
  Variable Integer Delay/1 -> AND/2
  Input/1 -> Variable Integer Delay/1, AND/1

== stateflow chart topology/Chart1 ==
  state standby
    du:
    du:
    out(1)=false;
    out(2)=false;
    out(3)=false;
    out(4)=false;
  state mode240
    du:
    out(1)=data(1);
    out(2)=data(2);
    out(3)=data(3);
    out(4)=data(4);
  state mode120
    du:
    out(1)=~data(1);
    out(2)=~data(2);
    out(3)=~data(3);
    out(4)=~data(4);
  (default) -> standby
  standby -> mode240 [order 1] : [mode ==  CHB_MODE.PFC240 || mode == CHB_MODE.INV240]
  mode240 -> standby : [mode ==  CHB_MODE.PFC120 || mode == CHB_MODE.INV120 ...
      | || mode ==  CHB_MODE.STANDBY]
  standby -> mode120 [order 2] : [mode ==  CHB_MODE.PFC120 || mode == CHB_MODE.INV120]
  mode120 -> standby : [mode ==  CHB_MODE.PFC240 || mode == CHB_MODE.INV240 ...
      | || mode ==  CHB_MODE.STANDBY]
  data: mode input Enum: CHB_MODE; data input boolean size=[1 4] =[1 4]; out output boolean size=[1 4]

== stateflow chart topology/Chart ==
  state standby
    du:
    du:
    out(1)=false;
    out(2)=false;
    out(3)=false;
    out(4)=false;
  state mode240
    du:
    out(1)=data(1);
    out(2)=data(2);
    out(3)=data(3);
    out(4)=data(4);
  state mode120
    du:
    out(1)=~data(1);
    out(2)=~data(2);
    out(3)=~data(3);
    out(4)=~data(4);
  (default) -> standby
  standby -> mode240 [order 1] : [mode ==  CHB_MODE.PFC240 || mode == CHB_MODE.INV240]
  mode240 -> standby : [mode ==  CHB_MODE.PFC120 || mode == CHB_MODE.INV120 ...
      | || mode ==  CHB_MODE.STANDBY]
  standby -> mode120 [order 2] : [mode ==  CHB_MODE.PFC120 || mode == CHB_MODE.INV120]
  mode120 -> standby : [mode ==  CHB_MODE.PFC240 || mode == CHB_MODE.INV240 ...
      | || mode ==  CHB_MODE.STANDBY]
  data: mode input Enum: CHB_MODE; data input boolean size=[1 4] =[1 4]; out output boolean size=[1 4]
